simulink model "ex1_sim"  (R2023b)
settings: Solver=FixedStepAuto  StartTime=0.0  StopTime=15  FixedStep=0.0001  RelTol=1e-3
InitFcn:
  | ex1
values from neighbouring files (symbols this model uses):
  N0 = 8    [ex1.m]    (also in ex2.m = 4)
  Nq = [(1 - 0.1) / (1 + 0.1), (1 - 0.2) / (1 + 0.2)]'    [ex1.m]    (also in ex2.m = [(1 - 0.26) / (1 + 0.26), (1 - 0.15) / (1 + 0.15), (1 - 0.17)
undefined symbols (not defined in the file or in its folder): A, C, F_A, F_B, F_E, F_F
settings Model: Creator=赵生  LastModifiedBy=赵生

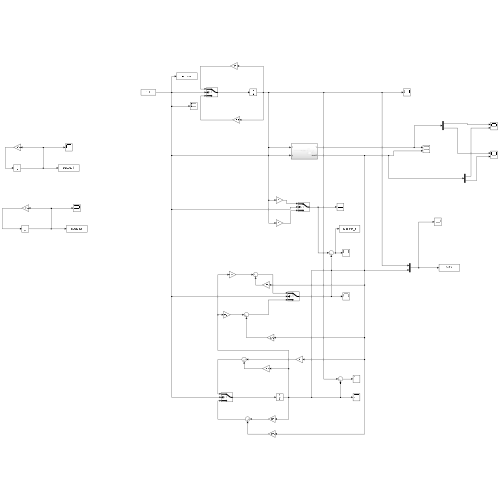
[thumbnail: Simulink's stored preview of the top-level diagram]
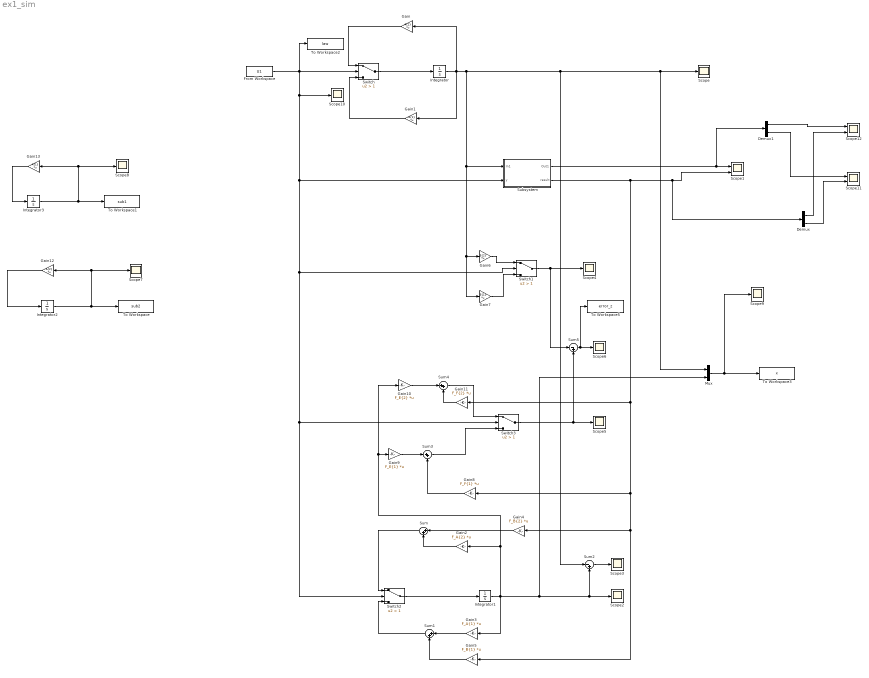
== system ex1_sim ==
  Demux : Demux  Outputs=2
  Demux1 : Demux  Outputs=2
  From Workspace : FromWorkspace  VariableName=U1
  Gain : Gain  Gain=A{2}  Multiplication=Matrix(K*u)
  Gain1 : Gain  Gain=A{1}  Multiplication=Matrix(K*u)
  Gain10 : Gain  Gain=F_E{2}  Multiplication=Matrix(K*u)
  Gain11 : Gain  Gain=F_F{2}  Multiplication=Matrix(K*u)
  Gain12 : Gain  Gain=A{2}  Multiplication=Matrix(K*u)
  Gain13 : Gain  Gain=A{1}  Multiplication=Matrix(K*u)
  Gain2 : Gain  Gain=F_A{2}  Multiplication=Matrix(K*u)
  Gain3 : Gain  Gain=F_A{1}  Multiplication=Matrix(K*u)
  Gain4 : Gain  Gain=F_B{2}  Multiplication=Matrix(K*u)
  Gain5 : Gain  Gain=F_B{1}  Multiplication=Matrix(K*u)
  Gain6 : Gain  Gain=E{2}  Multiplication=Matrix(K*u)
  Gain7 : Gain  Gain=E{1}  Multiplication=Matrix(K*u)
  Gain8 : Gain  Gain=F_F{1}  Multiplication=Matrix(K*u)
  Gain9 : Gain  Gain=F_E{1}  Multiplication=Matrix(K*u)
  Integrator : Integrator  InitialCondition=[6 7]'
  Integrator1 : Integrator  InitialCondition=[8 9]'
  Integrator2 : Integrator  InitialCondition=[6 7]'
  Integrator3 : Integrator  InitialCondition=[6 7]'
  Mux : Mux  Inputs=2
  Scope{,2..10} (10 alike) : Scope
  Scope1 : Scope  NumInputPorts=2
  Scope11 : Scope  NumInputPorts=2
  Scope12 : Scope  NumInputPorts=2
  Subsystem : Subsystem
  Sum{,1,3..4} (4 alike) : Sum  Inputs=|++
  Sum2 : Sum  Inputs=|-+
  Sum5 : Sum  Inputs=|-+
  Switch{,1..3} (4 alike) : Switch  Criteria=u2 > Threshold  Threshold=1  SaturateOnIntegerOverflow=off  InputSameDT=off
  To Workspace : ToWorkspace  VariableName=sub2  SaveFormat=Structure With Time  SampleTime=-1
  To Workspace1 : ToWorkspace  VariableName=sub1  SaveFormat=Structure With Time  SampleTime=-1
  To Workspace2 : ToWorkspace  VariableName=law  SaveFormat=Structure With Time  SampleTime=-1
  To Workspace3 : ToWorkspace  VariableName=x  SaveFormat=Structure With Time  SampleTime=-1
  To Workspace5 : ToWorkspace  VariableName=error_z  SaveFormat=Structure With Time  SampleTime=-1
  wires:
  Switch/1 -> Integrator/1
  Integrator/1 -> Mux/1, Scope/1, Sum2/1, Subsystem/1(In1), Gain7/1, Gain6/1, Gain/1, Gain1/1
  Gain/1 -> Switch/1
  Gain1/1 -> Switch/3
  Subsystem/1(Out1) -> Demux1/1, Scope1/1
  Subsystem/2(result) -> Demux/1, Scope1/2, Gain11/1, Gain8/1, Gain4/1, Gain5/1
  Switch2/1 -> Integrator1/1
  Gain2/1 -> Sum/2
  Integrator1/1 -> Gain9/1, Gain10/1, Gain2/1, Scope2/1, Sum2/2, Mux/2, Gain3/1
  Gain4/1 -> Sum/1
  Sum/1 -> Switch2/1
  Gain3/1 -> Sum1/1
  Gain5/1 -> Sum1/2
  Sum1/1 -> Switch2/3
  Sum2/1 -> Scope3/1
  Gain6/1 -> Switch1/1
  Gain7/1 -> Switch1/3
  Switch1/1 -> Sum5/1, Scope4/1
  Gain8/1 -> Sum3/2
  Sum3/1 -> Switch3/3
  Gain9/1 -> Sum3/1
  Gain10/1 -> Sum4/1
  Sum4/1 -> Switch3/1
  Gain11/1 -> Sum4/2
  Switch3/1 -> Scope5/1, Sum5/2
  Sum5/1 -> Scope6/1, To Workspace5/1
  Integrator2/1 -> To Workspace/1, Scope7/1, Gain12/1
  Gain12/1 -> Integrator2/1
  Integrator3/1 -> To Workspace1/1, Gain13/1, Scope8/1
  Gain13/1 -> Integrator3/1
  Mux/1 -> Scope9/1, To Workspace3/1
  From Workspace/1 -> To Workspace2/1, Scope10/1, Switch1/2, Switch2/2, Switch3/2, Subsystem/2(y), Switch/2
  Demux1/2 -> Scope11/1
  Demux/2 -> Scope11/2
  Demux1/1 -> Scope12/1
  Demux/1 -> Scope12/2

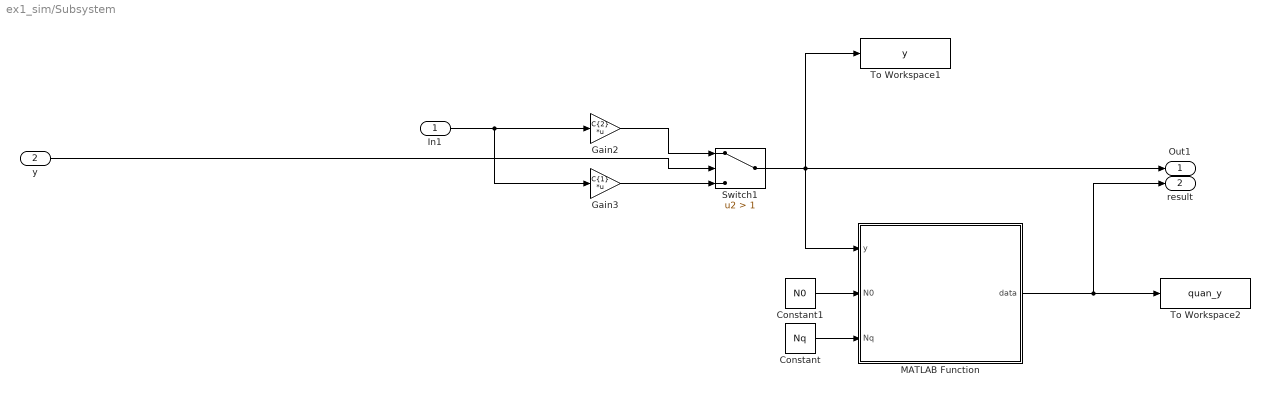
== system ex1_sim/Subsystem ==
  In1 : Inport
  y : Inport  Port=2
  Constant : Constant  Value=Nq
  Constant1 : Constant  Value=N0
  Gain2 : Gain  Gain=C{2}  Multiplication=Matrix(K*u)
  Gain3 : Gain  Gain=C{1}  Multiplication=Matrix(K*u)
  MATLAB Function : MATLAB Function  TreatAsAtomicUnit=on
  Switch1 : Switch  Criteria=u2 > Threshold  Threshold=1  SaturateOnIntegerOverflow=off  InputSameDT=off
  To Workspace1 : ToWorkspace  VariableName=y  SaveFormat=Structure With Time  SampleTime=-1
  To Workspace2 : ToWorkspace  VariableName=quan_y  SaveFormat=Structure With Time  SampleTime=-1
  Out1 : Outport
  result : Outport  Port=2
  wires:
  Switch1/1 -> To Workspace1/1, Out1/1, MATLAB Function/1(y)
  MATLAB Function/1(data) -> To Workspace2/1, result/1
  Gain3/1 -> Switch1/3
  In1/1 -> Gain3/1, Gain2/1
  Constant/1 -> MATLAB Function/3(Nq)
  Gain2/1 -> Switch1/1
  Constant1/1 -> MATLAB Function/2(N0)
  y/1 -> Switch1/2

== matlab function ex1_sim/Subsystem/MATLAB Function ==
  data: y input; N0 input; data output; Nq input
function data = quantize_2d(y, N0, Nq)
data = zeros(size(y));
for c = 1:2
    yc = y(c, :);
    aleph = Nq(c);
    psi0 = N0;
    idx = yc > 0;
    if any(idx) 
        phi = ceil(log(yc(idx) / (psi0 * (1 + aleph) / 2)) / log(aleph));
        data(c, idx) = (aleph.^phi) * psi0;
    end
end
